simulink model "Robot_Control"  (R2023b)
settings: Solver=FixedStepDiscrete  StartTime=0.0  StopTime=inf  FixedStep=t_sample  RelTol=1e-3
undefined symbols (not defined in the file): t_sample
settings Model: Creator=FIRSTMentor  LastModifiedBy=ander
settings OptimizationCC: DefaultParameterBehavior=Inlined  StrengthReduction=on  PassReuseOutputArgsAs=Individual arguments  ZeroExternalMemoryAtStartup=off  ZeroInternalMemoryAtStartup=off  OptimizeBlockOrder=speed  OptimizationPriority=Speed  OptimizationCustomize=off  MultiThreadedLoops=on  EfficientTunableParamExpr=on
settings DebuggingCC: MergeDetectMultiDrivingBlocksExec=none  ParameterTunabilityLossMsg=error
settings HardwareCC: ProdBitPerPointer=32  ProdBitPerSizeT=32  ProdBitPerPtrDiffT=32  ProdLargestAtomicInteger=Long  ProdWordSize=32  ProdHWDeviceType=ARM Compatible->ARM 7
settings ModelReferenceCC: PropagateSignalLabelsOutOfModel=off
settings SFSimCC: MATLABDynamicMemAlloc=off
settings RTWCC: Description=Embedded Coder  SystemTargetFile=ert.tlc  GenCodeOnly=on  TemplateMakefile=ert_default_tmf  Toolchain=MinGW64 | gmake (64-bit Windows)
settings CodeAppCC: ForceParamTrailComments=on  IgnoreCustomStorageClasses=off  OperatorAnnotations=on  SimulinkDataObjDesc=on  SFDataObjDesc=on  InsertBlockDesc=on
settings ERTTargetCC: TargetLangStandard=C99 (ISO)  UtilityFuncGeneration=Shared location  SupportVariableSizeSignals=on  ParenthesesLevel=Maximum  InlinedParameterPlacement=NonHierarchical  ERTCustomFileTemplate=example_file_process.tlc

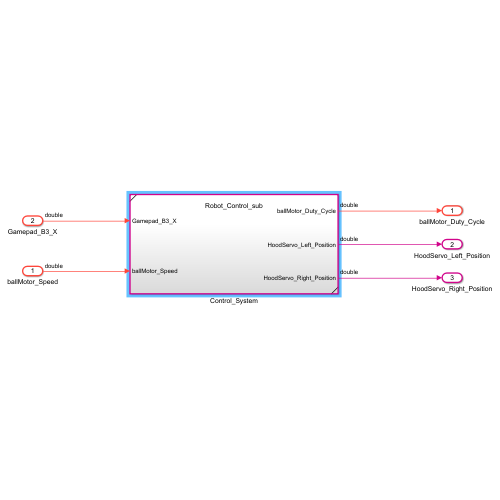
[thumbnail: Simulink's stored preview of the top-level diagram]
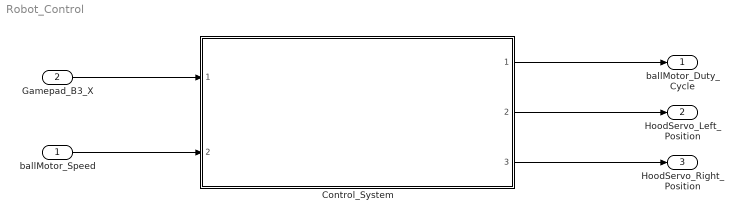
== system Robot_Control ==
  ballMotor_Speed : Inport
  Gamepad_B3_X : Inport  Port=2
  Control_System : Subsystem  SystemSampleTime=t_sample  RTWFcnName=Model_Step  ReferencedSubsystem=Robot_Control_sub
      settings: RTWSystemCode=Nonreusable function  RTWFcnNameOpts=User specified
  ballMotor_Duty_Cycle : Outport
  HoodServo_Left_Position : Outport  Port=2
  HoodServo_Right_Position : Outport  Port=3
  wires:
  Control_System/1 -> ballMotor_Duty_Cycle/1
  ballMotor_Speed/1 -> Control_System/2
  Gamepad_B3_X/1 -> Control_System/1
  Control_System/2 -> HoodServo_Left_Position/1
  Control_System/3 -> HoodServo_Right_Position/1
